simulink model "sm_wheel_loader_test_CG"  (R2025a)
settings: Solver=VariableStepAuto  StartTime=0.0  StopTime=1e-4  RelTol=1e-3  AbsTol=1e-3  EnableMultiTasking=on
InitFcn:
  | if(exist('cg_loc'))
  |     cg_offset = cg_loc.Data;
  | else
  |     cg_offset = [0 0 0];
  | end
undefined symbols (not defined in the file or in its folder): X, Y, Z
libraries: sm_lib x6, fl_lib x6, nesl_utility x4, sm_wheel_loader_lib x2, simulink x1
Description:
  | Wheel Loader Chassis CG Check
  | Copyright 2023-2025 The MathWorks, Inc.
settings Model: Creator=smiller  LastModifiedBy=smiller
settings SolverCC: AutoScaleAbsTol=off  AlgebraicLoopSolver=TrustRegion  MaxZcPerStep=1.0
settings DataIOCC: LimitDataPoints=on  MaxDataPoints=10000  ReturnWorkspaceOutputs=off
settings OptimizationCC: ReuseModelBlockBuffer=off  LifeSpan=inf
settings DebuggingCC: UnconnectedInputMsg=warning  UnconnectedOutputMsg=warning  UnconnectedLineMsg=warning  AllowSymbolicDim=off  SubsystemReferenceDiagnosticForUnitTest=warning  SFUnexpectedBacktrackingDiag=warning  SFNoUnconditionalDefaultTransitionDiag=warning  SFExecutionAtInitializationDiag=none  ArithmeticOperatorsInVariantConditions=warning
settings ModelReferenceCC: EnableRefExpFcnMdlSchedulingChecks=on
settings SFSimCC: SimUseLocalCustomCode=off  CustomCodeUndefinedFunction=UseInterfaceOnly
settings RTWCC: RTWUseLocalCustomCode=off  GPUComputeCapability=3.5  DLArmComputeVersion=19.05
settings CodeAppCC: StateflowObjectComments=on
settings GRTTargetCC: TargetLangStandard=C89/C90 (ANSI)
settings ConfigComp: CovMetricSettings=dw  CovSaveCumulativeToWorkspaceVar=on  CovSaveSingleToWorkspaceVar=on  CovExternalEMLEnable=off  CovSFcnEnable=off
settings SimscapeCC: SimscapeLogType=all  SimscapeLogSimulationStatistics=on  SimscapeLogDataHistory=10000.0
settings DiagnosticsConfigSet: SimMechanicsUnconnectedFramePorts=none  SimMechanicsConflictingReferenceFrames=none
settings ExplorerConfigSet: InternalSimMechanicsExplorerSettings="<ExplorerConfiguration><canonicalview>default</canonicalview><AnimationSetting><BasePlaybackSpeed>1.0</BasePlaybackSpeed><PlaybackSpeedFactor>1.0</PlaybackSpeedFactor></AnimationSetting><TilePanel><TileInfo><Tiles Columns=\"1\" Count=\"1\" Rows=\"1\"><Column Weight=\"1\"/><Row Weight=\"1\"/><Tile Height=\"1\" Width=\"1\" X=\"0\" Y=\"0\"/></Tiles></TileInfo><SceneInfo><SceneViewer><BGColor><R>1</R><G>1</G><B>1</B></BGColor><Camera><DoPerspective>off</DoPerspective><Position><X>-0.214259147644042969</X><Y>-5.87822117757797269</Y><Z>1.17845511436462358</Z></Position><Center><X>-0.214259147644042969</X><Y>-1.98409333229064888</Y><Z>1.17845511436462358</Z></Center><Up><X>0</X><Y>-0</Y><Z>1</Z></Up><ViewLimDist>1</ViewLimDist><YLim>1.89117988823481986</YLim><XLim>2.78582895994186419</XLim></Camera></SceneViewer></SceneInfo></TilePanel><MechEditorPanel><Cameras/><GfxPanelCameraMap/><VideoCreator><PlaybackSpeedRatio>1.0</PlaybackSpeedRatio><FrameRate>30</FrameRate><VideoFormat>Motion JPEG AVI</VideoFormat><FrameSize>auto</FrameSize></VideoCreator></MechEditorPanel></ExplorerConfiguration>"

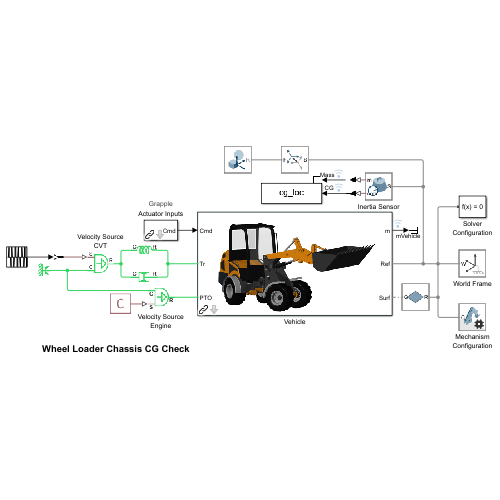
[thumbnail: Simulink's stored preview of the top-level diagram]
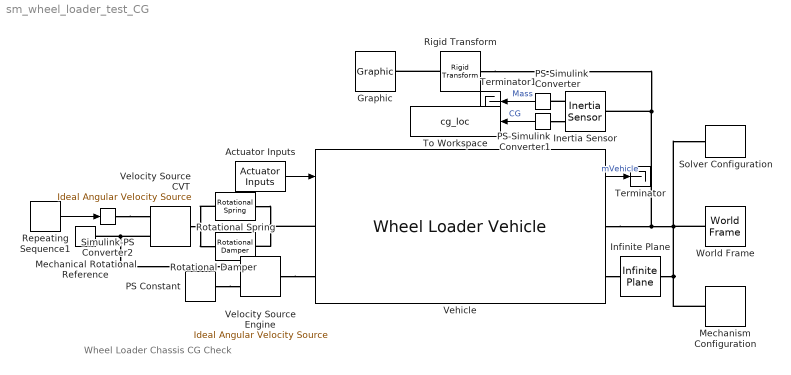
== system sm_wheel_loader_test_CG ==
  note: Wheel Loader Chassis CG Check
  Actuator Inputs : sm_wheel_loader_lib/Actuator Inputs  popup_steering=on  popup_linkage=on  popup_impl=Grapple
      settings: AttributesFormatString=%<popup_impl>
  Graphic : sm_lib/Body Elements/Graphic  GraphicType=Marker  MarkerShape=Cube  MarkerSize=10  GraphicVisPropType=SimpleVisualProperties  GraphicDiffuseColor=[1 0 0]  GraphicOpacity=1.0  GraphicSpecularColor=[0.5 0.5 0.5 1.0]  GraphicAmbientColor=[0.15 0.15 0.15 1.0]  GraphicEmissiveColor=[0.0 0.0 0.0 1.0]  GraphicShininess=75
  Inertia Sensor : sm_lib/Body Elements/Inertia Sensor  SensorExtent=Mechanism  SpanWeldJoints=off  ExcludeGroundedBodies=on  MeasurementFrame=Attached  SenseMass=on  SenseCenterOfMass=on  SenseInertiaMatrix=off  SenseCenteredInertiaMatrix=off  SensePrincipalInertiaMatrix=off  SenseRotationMatrix=off  GraphicType=None  PrincipalInertiaFrameSize=20  GraphicVisPropType=SimpleVisualProperties  GraphicDiffuseColor=[0.5 0.5 0.5]  GraphicOpacity=1.0  GraphicSpecularColor=[0.5 0.5 0.5 1.0]  GraphicAmbientColor=[0.15 0.15 0.15 1.0]  GraphicEmissiveColor=[0.0 0.0 0.0 1.0]  GraphicShininess=75
  Infinite Plane : sm_lib/Curves and Surfaces/Infinite Plane  GraphicType=Rectangle  GraphicPlaneWidth=1  GraphicPlaneWidthUnits=m  GraphicPlaneHeight=1  GraphicPlaneHeightUnits=m  GraphicVisPropType=SimpleVisualProperties  GraphicDiffuseColor=[0.5 0.5 0.5]  GraphicOpacity=0.25  GraphicSpecularColor=[0.5 0.5 0.5 1.0]  GraphicAmbientColor=[0.15 0.15 0.15 1.0]  GraphicEmissiveColor=[0.0 0.0 0.0 1.0]  GraphicShininess=75
  Mechanical Rotational Reference : fl_lib/Mechanical/Rotational Elements/Mechanical Rotational Reference
  Mechanism Configuration : sm_lib/Utilities/Mechanism Configuration  UniformGravity=Constant  GravityVector=[0 0 -9.80665]  GravityVectorUnits=m/s^2  LinearizationDelta=0.001  JointModeTransitionNonlinearIterations=2
  PS Constant : fl_lib/Physical Signals/Sources/PS Constant  constant=HMPST.Eng.wTarget rpm
  PS-Simulink Converter : nesl_utility/PS-Simulink Converter  PhysicalDomain=network_engine_domain  SubClassName=ps_output  LeftPortType=input  RightPortType=output  PseudoPeriodic=off  Frequencies=[]  VectorFormat=inherit  Unit=inherit  AffineConversion=off
  PS-Simulink Converter1 : nesl_utility/PS-Simulink Converter  PhysicalDomain=network_engine_domain  SubClassName=ps_output  LeftPortType=input  RightPortType=output  PseudoPeriodic=off  Frequencies=[]  VectorFormat=inherit  Unit=inherit  AffineConversion=off
  Repeating Sequence1 : simulink/Sources/Repeating Sequence  rep_seq_t=[0 10.2 12 15 17.1 32.3 33.1 36.2 38.9 41.0 43 46 48 62.9 65 68 70]  rep_seq_y=[0 0 1 1 0 0 -1 -1 0 0 1 1 0 0 -1 -1 0]*1160
  Rigid Transform : sm_lib/Frames and Transforms/Rigid Transform  RotationMethod=None  FollAlignAxisA=+X  BaseAlignAxisA=+Y  FollAlignAxisB=+Y  BaseAlignAxisB=+Z  RotationStandardAxis=+Z  RotationAngle=0.0  RotationAngleUnits=deg  RotationArbitraryAxis=[0 0 1]  RotationSequenceAxes=FollowerAxes  RotationSequence=XYX  RotationSequenceAngles=[0 0 0]  RotationSequenceAnglesUnits=deg  RotationMatrix=[1 0 0; 0 1 0; 0 0 1]  Quaternion=[1 0 0 0]  TranslationMethod=Cartesian  TranslationCartesianOffset=cg_offset  TranslationCartesianOffsetUnits=m  TranslationStandardAxis=+Z  TranslationStandardOffset=0  TranslationStandardOffsetUnits=m  TranslationROffset=0  TranslationROffsetUnits=m  TranslationThetaOffset=0  TranslationThetaOffsetUnits=deg  TranslationZOffset=0  TranslationZOffsetUnits=m
  Rotational Damper : fl_lib/Mechanical/Rotational Elements/Rotational Damper  D=5 N*m*s/rad  w_specify=off  w_priority=None  w=0 rad/s  w_nominal_specify=off  w_nominal_value=1  w_nominal_unit=rad/s  t_specify=off  t_priority=None  t=0 N*m  t_nominal_specify=off  t_nominal_value=1  t_nominal_unit=N*m
  Rotational Spring : fl_lib/Mechanical/Rotational Elements/Rotational Spring  spr_rate=1000 N*m/rad  w_specify=off  w_priority=None  w=0 rad/s  w_nominal_specify=off  w_nominal_value=1  w_nominal_unit=rad/s  t_specify=off  t_priority=None  t=0 N*m  t_nominal_specify=off  t_nominal_value=1  t_nominal_unit=N*m  phi_specify=off  phi_priority=High  phi=0 rad  phi_nominal_specify=off  phi_nominal_value=1  phi_nominal_unit=rad
  Simulink-PS Converter2 : nesl_utility/Simulink-PS Converter  PhysicalDomain=network_engine_domain  SubClassName=ps_input  LeftPortType=input  RightPortType=output  PseudoPeriodic=off  Frequencies=[]  NoiseDistribution=none  NoiseParameters=[]  Unit=rpm  AffineConversion=off  FilteringAndDerivatives=filter  SimscapeFilterOrder=2  InputFilterTimeConstant=0.1  UdotUserProvided=0
  Solver Configuration : nesl_utility/Solver Configuration  PhysicalDomain=network_engine_domain  SubClassName=solver  LeftPortType=input  RightPortType=generic  Tones=[]  Harmonics=[]  SimulateNoise=off  Profile=off  UseLocalSampling=off  EnableSwitchedLinearOptims=on  FrequencyDomain=off  UseCCode=off  RelTol=0.001  AbsTol=1e-06  MinStep=1e-09  ToWorkspace=off  RevertToSquareIcSolve=off  NumHomotopyIterations=100  PhasorMode=off  PhasorModeNumHarmonics=1  ConsistencySolver=NEWTON_XTOL_AFTER_FTOL  IndexReductionMethod=DerivativeReplacement  DoDC=off  ResidualTolerance=1e-09  ConsistencyTolSource=GLOBAL  ConsistencyAbsTol=0.001  ConsistencyRelTol=0.001  ConsistencyTolFactor=0.001  UseLocalSolver=off  LocalSolverChoice=NE_BACKWARD_EULER_ADVANCER  ResolveIndetEquations=on  FunctionEvalNumThread=1  LocalSolverSampleTime=0.001  DoFixedCost=off  MaxNonlinIter=3  MaxModeIter=2  ComputeImpulses=off  ImpulseIterations=2  LinearAlgebra=Sparse  LinearAlgebraNumThread=0  EquationFormulation=NE_TIME_EF  DelaysMemoryBudget=1024  AutomaticFiltering=on  FilteringTimeConstant=0.001  PartitionStorageMethod=AS_NEEDED  PartitionMemoryBudget=1024  PartitionMethod=FAST  MultibodyUseLocalSolver=off  MultibodyLocalSolverChoice=ODE1  MultibodyLocalSolverSampleTime=0.001
  Terminator : Terminator
  Terminator1 : Terminator
  To Workspace : ToWorkspace  VariableName=cg_loc  SaveFormat=Timeseries  SampleTime=-1
      settings: MaxDataPoints=1
  Vehicle : sm_wheel_loader_lib/Wheel Loader Vehicle  VariantControl=simVariant == 1  popup_impl=Bucket  popup_actuator_model=Ideal  popup_load=None  popup_driveline_model=Driveline 3D  popup_driveJointF=U Joint  popup_driveJointR=U Joint  popup_contact=Sphere
  Velocity Source CVT : fl_lib/Mechanical/Mechanical Sources/Ideal Angular Velocity Source
  Velocity Source Engine : fl_lib/Mechanical/Mechanical Sources/Ideal Angular Velocity Source
  World Frame : sm_lib/Frames and Transforms/World Frame
  wires:
  Actuator Inputs/1 -> Vehicle/1
  PS-Simulink Converter1/1 -> To Workspace/1  "CG"
  PS-Simulink Converter/1 -> Terminator1/1  "Mass"
  Vehicle/1 -> Terminator/1  "mVehicle"
  Repeating Sequence1/1 -> Simulink-PS Converter2/1
  connections:
  World Frame/RConn1 -- Inertia Sensor/LConn1 -- Rigid Transform/LConn1 -- Vehicle/RConn1 -- Mechanism Configuration/RConn1 -- Infinite Plane/LConn1 -- Solver Configuration/RConn1
  Velocity Source Engine/LConn1 -- Vehicle/LConn2
  Vehicle/RConn2 -- Infinite Plane/RConn1
  Inertia Sensor/RConn1 -- PS-Simulink Converter/LConn1
  PS-Simulink Converter1/LConn1 -- Inertia Sensor/RConn2
  Rotational Damper/LConn1 -- Vehicle/LConn1 -- Rotational Spring/LConn1
  Rotational Damper/RConn1 -- Rotational Spring/RConn1 -- Velocity Source CVT/LConn1
  Velocity Source CVT/RConn2 -- Velocity Source Engine/RConn2 -- Mechanical Rotational Reference/LConn1
  Simulink-PS Converter2/RConn1 -- Velocity Source CVT/RConn1
  PS Constant/RConn1 -- Velocity Source Engine/RConn1
  Rigid Transform/RConn1 -- Graphic/RConn1
